simulink model "PLL"  (R2023a)
settings: Solver=FixedStepDiscrete  StartTime=0.0  StopTime=100e-6  FixedStep=25e-12  RelTol=1e-3
model workspace (MAT data in the model file):
  R = 1000
undefined symbols (not defined in the file): DiscIntNeverNeededParam
libraries: simulink_extras x2, simulink x1
settings Model: Creator=mazen  LastModifiedBy=mazen
settings OptimizationCC: BlockReduction=off  ConditionallyExecuteInputs=off  DefaultParameterBehavior=Inlined  OptimizeBlockIOStorage=off  EnhancedBackFolding=on  PassReuseOutputArgsThreshold=0  OptimizeBlockOrder=speed  DifferentSizesBufferReuse=on
settings DebuggingCC: ParameterTunabilityLossMsg=error
settings HardwareCC: TargetBitPerPointer=64  TargetBitPerSizeT=64  TargetBitPerPtrDiffT=64  TargetLongLongMode=on  TargetIntDivRoundTo=Zero  TargetEndianess=LittleEndian  TargetWordSize=64  TargetHWDeviceType=Generic->Custom  ProdEqTarget=off
settings SFSimCC: MATLABDynamicMemAlloc=off
settings RTWCC: Description=SystemVerilog DPI Component Generator  SystemTargetFile=systemverilog_dpi_grt.tlc  TemplateMakefile=systemverilog_dpi_grt_default_tmf
settings CodeAppCC: ForceParamTrailComments=on  MaxIdLength=256  OperatorAnnotations=on
settings DPIGRTTargetCC: TargetFcnLib=ansi_tfl_table_tmw.mat  GenFloatMathFcnCalls=NOT IN USE  TargetLangStandard=C99 (ISO)  CodeReplacementLibrary=None  UtilityFuncGeneration=Auto  MultiwordTypeDef=System defined  MultiwordLength=2048  DynamicStringBufferSize=256  GenerateFullHeader=on  InferredTypesCompatibility=off  GenerateSampleERTMain=off  GenerateTestInterfaces=off  ModelReferenceCompliant=on  ParMdlRefBuildCompliant=on  CompOptLevelCompliant=off  ConcurrentExecutionCompliant=off  IncludeMdlTerminateFcn=on  CombineOutputUpdateFcns=off  CombineSignalStateStructs=on  GroupInternalDataByFunction=off  SuppressErrorStatus=off  IncludeFileDelimiter=Auto  ERTCustomFileBanners=off  SupportAbsoluteTime=on  LogVarNameModifier=rt_  MatFileLogging=off  CodeInterfacePackaging=Reusable function  PurelyIntegerCode=off  SupportNonFinite=on  SupportComplex=on  SupportContinuousTime=on  SupportNonInlinedSFcns=on  RemoveDisableFunc=off  RemoveResetFunc=off  SupportVariableSizeSignals=off  ParenthesesLevel=Nominal  CastingMode=Nominal  MATLABClassNameForMDSCustomization=Simulink.SoftwareTarget.TargetSpecificTriggerConfigurationBase  ModelStepFunctionPrototypeControlCompliant=off  CPPClassGenCompliant=off  AutosarCompliant=off  MDXCompliant=off  GRTInterface=off  GenerateAllocFcn=on  UseToolchainInfoCompliant=on  GenerateSharedConstants=on  CoderGroups=[]  AccessMethods=[]  LookupTableObjectStructAxisOrder=1,2,3,4,...  LUTObjectStructOrderExplicitValues=Size,Breakpoints,Table  LUTObjectStructOrderEvenSpacing=Size,Breakpoints,Table  ArrayLayout=Column-major  UnsupportedSFcnMsg=error  ERTHeaderFileRootName=$R$E  ERTSourceFileRootName=$R$E  ERTDataFileRootName=$R_data  OptimizeReductions=off  RTWCAPISignals=on  RTWCAPIParams=off  RTWCAPIStates=off  RTWCAPIRootIO=off  ExtMode=off  ExtModeTransport=0  ExtModeStaticAlloc=off  ExtModeStaticAllocSize=1000000  ExtModeTesting=off  ExtModeMexFile=ext_comm  GenerateASAP2=off  MultiInstanceErrorCode=Error  DPICustomizeSystemVerilogCode=off  DPISystemVerilogTemplate=svdpi_event.vgt  DPIReportRunTimeError=off  DPIRunTimeErrorSeverity=Fatal  DPIScalarizePorts=off  DPIGenerateTestBench=off  DPITestBenchSimulator=Mentor Graphics Questasim  DPITestPointAccessFcnInterface=None  DPIFixedPointDataType=CompatibleCType  DPIPortConnection=Port list  DPICompositeDataType=Flattened  DPIComponentTemplateType=Sequential

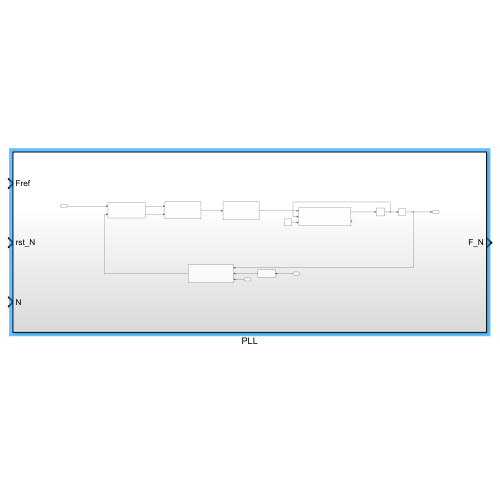
[thumbnail: Simulink's stored preview of the top-level diagram]
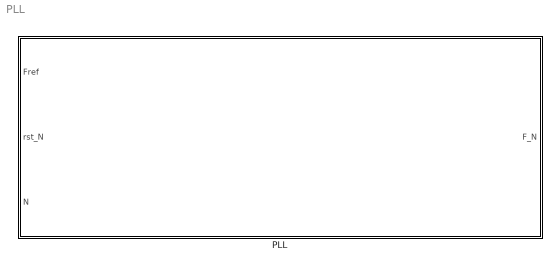
== system PLL ==
  PLL : Subsystem

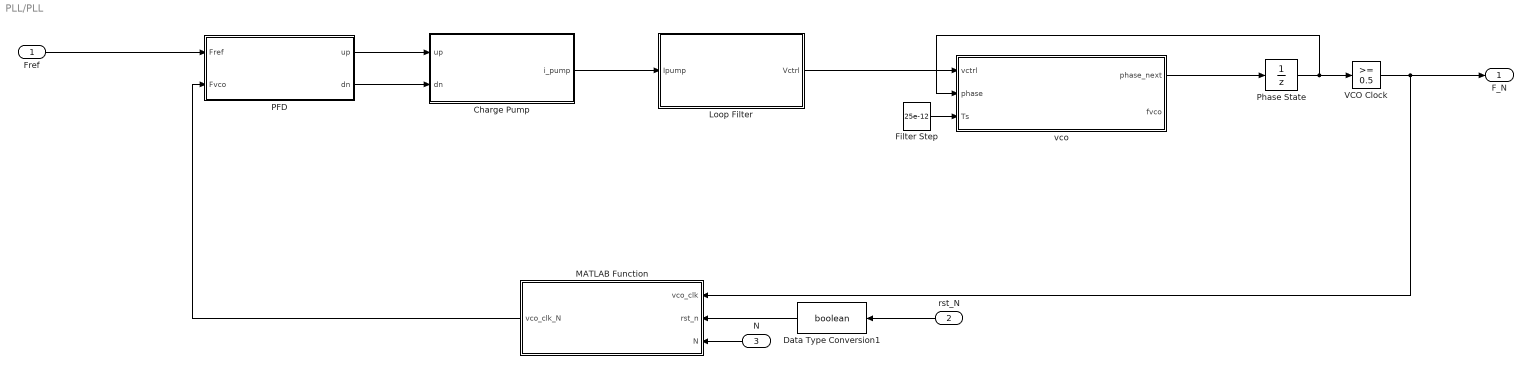
== system PLL/PLL ==
  Fref : Inport  OutDataTypeStr=boolean
  rst_N : Inport  Port=2  OutDataTypeStr=boolean
  N : Inport  Port=3  OutDataTypeStr=double
  Charge Pump : MATLAB Function  TreatAsAtomicUnit=on
  Data Type Conversion1 : DataTypeConversion  OutDataTypeStr=boolean  SaturateOnIntegerOverflow=off  RndMeth=Floor
  Filter Step : Constant  Value=25e-12
  Loop Filter : Subsystem
  MATLAB Function : MATLAB Function  TreatAsAtomicUnit=on
  PFD : Subsystem
  Phase State : UnitDelay  SampleTime=25e-12  HasFrameUpgradeWarning=on
  VCO Clock : simulink/Logic and Bit Operations/Compare To Constant  relop=>=  const=0.5  OutDataTypeStr=boolean
  vco : MATLAB Function  TreatAsAtomicUnit=on
  F_N : Outport  OutDataTypeStr=boolean
  wires:
  N/1 -> MATLAB Function/3(N)
  Data Type Conversion1/1 -> MATLAB Function/2(rst_n)
  PFD/2(dn) -> Charge Pump/2(dn)
  PFD/1(up) -> Charge Pump/1(up)
  VCO Clock/1 -> MATLAB Function/1(vco_clk), F_N/1
  Phase State/1 -> VCO Clock/1, vco/2(phase)
  Filter Step/1 -> vco/3(Ts)
  vco/1(phase_next) -> Phase State/1
  rst_N/1 -> Data Type Conversion1/1
  Loop Filter/1(Vctrl) -> vco/1(vctrl)
  Charge Pump/1(i_pump) -> Loop Filter/1(Ipump)
  Fref/1 -> PFD/1(Fref)
  MATLAB Function/1(vco_clk_N) -> PFD/2(Fvco)

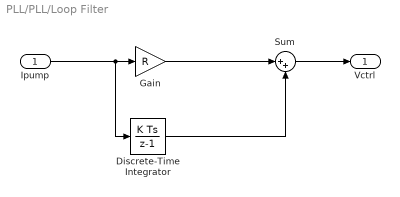
== system PLL/PLL/Loop Filter ==
  Ipump : Inport
  Discrete-Time Integrator : DiscreteIntegrator  gainval=1 / 10e-12  InitialCondition=0.5  SampleTime=25e-12  ICPrevOutput=DiscIntNeverNeededParam  ICPrevScaledInput=DiscIntNeverNeededParam
  Gain : Gain  Gain=R
  Sum : Sum  Inputs=|++
  Vctrl : Outport
  wires:
  Discrete-Time Integrator/1 -> Sum/2
  Gain/1 -> Sum/1
  Ipump/1 -> Discrete-Time Integrator/1, Gain/1
  Sum/1 -> Vctrl/1

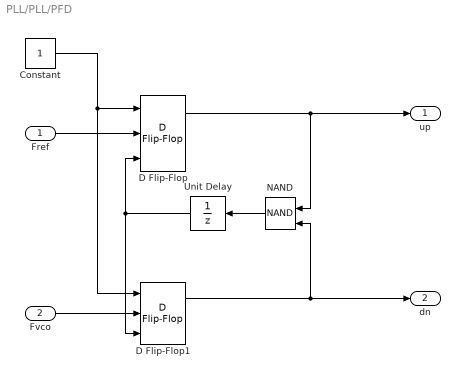
== system PLL/PLL/PFD ==
  Fref : Inport
  Fvco : Inport  Port=2
  Constant : Constant  OutDataTypeStr=boolean
  D Flip-Flop : simulink_extras/Flip Flops/D Flip-Flop
  D Flip-Flop1 : simulink_extras/Flip Flops/D Flip-Flop
  NAND : Logic  Operator=NAND  IconShape=distinctive  AllPortsSameDT=off  OutDataTypeStr=boolean
  Unit Delay : UnitDelay  SampleTime=-1  HasFrameUpgradeWarning=on
  up : Outport
  dn : Outport  Port=2
  wires:
  Fvco/1 -> D Flip-Flop1/2
  Fref/1 -> D Flip-Flop/2
  Constant/1 -> D Flip-Flop1/1, D Flip-Flop/1
  NAND/1 -> Unit Delay/1
  D Flip-Flop/1 -> NAND/1, up/1
  D Flip-Flop1/1 -> dn/1, NAND/2
  Unit Delay/1 -> D Flip-Flop1/3, D Flip-Flop/3

== matlab function PLL/MATLAB Function ==
  data: vco_clk input; vco_clk_N output; rst_n input; N input
function vco_clk_N = freq_divider(vco_clk, rst_n, N)
%#codegen

persistent prevClk count periodCycles fracAccum clkOut

if isempty(prevClk)
    prevClk      = false;
    count        = 0;
    periodCycles = 0;
    fracAccum    = 0;
    clkOut       = false;
end

clk = vco_clk > 0;
rise = clk && ~prevClk;
prevClk = clk;

if ~rst_n
    count        = 0;
    periodCycles = 0;
    fracAccum    = 0;
    clkOut       = false;
elseif rise
    if count == 0
        % Choose the length of the next full feedback period.
        baseCycles = floor(double(N));
        fracAccum = fracAccum + (double(N) - baseCycles);

        extraCycle = floor(fracAccum);
        periodCycles = baseCycles + extraCycle;
        fracAccum = fracAccum - extraCycle;
    end

    clkOut = count < floor(periodCycles / 2);

    count = count + 1;
    if count == periodCycles
        count = 0;
    end
end

vco_clk_N = clkOut;
end

== matlab function PLL/Charge Pump ==
  data: up input; i_pump output; dn input
function i_pump = charge_pump(up, dn)
i_pump = 100e-6 * (double(up) - double(dn));
end

== matlab function PLL/vco ==
  data: vctrl input; phase_next output; phase input; Ts input; fvco output
function [phase_next, fvco] = vco_model(vctrl, phase, Ts)
fvco = 95e6 + 50e6 * (vctrl - 0.5);
phase_next = mod(phase + fvco * Ts, 1);
end
